simulink model "PV_Subsystem"  (R2024b)
settings: Solver=VariableStepAuto  StartTime=0.0  StopTime=10.0  RelTol=1e-3
libraries: spsSeriesRLCBranchLib x3, spsVoltageMeasurementLib x2, spsCurrentMeasurementLib x1, spsDiodeLib x1, spsIGBTDiodeLib x1, spsPVArrayLib x1, spsPWMGeneratorDCDCLib x1, sps_lib x1
settings Model: Creator=Raju  LastModifiedBy=Raju

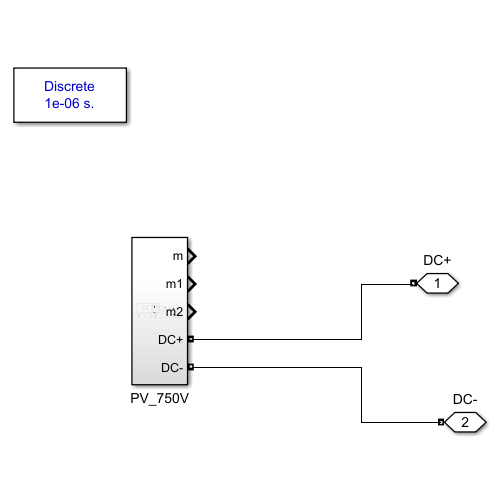
[thumbnail: Simulink's stored preview of the top-level diagram]
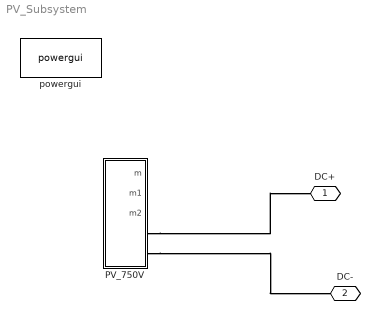
== system PV_Subsystem ==
  PV_750V : Subsystem
  powergui : sps_lib/powergui  Priority=1  SimulationMode=Discrete  SampleTime=1e-6  frequency=60  Iterations=50  frequencyindice=0  Pbase=100e6  ErrMax=1e-4  UnitsV=kV  UnitsW=MW  buscounter=0  FunctionMessages=off  echomessages=off  EnableUseOfTLC=off  CurrentSourceSwitches=off  DisableSnubberDevices=off  DisableRonSwitches=off  DisableVfSwitches=off  DisplayEquations=off  AutomaticDiscreteSolvers=off  SolverType=Tustin/Backward Euler (TBE)  Interpol=off  ExternalGateDelay=off  methode=off  Ts=100  x0status=blocks  SPID=on  SwTol=0  HookPort=off  NonlinearTolerance=1e-4  nMaxIteration=100  ContinueOnMaxIteration=off  RestoreLinks=warning  ResistiveCurrentMeasurement=off  Frange=[0:2:500]  Ylog=off  Xlog=on  ShowGrid=off  save=off  variable=ZData  structure=0  ZoomFFT=off  StartTime=0.0  cycles=1  DisplayStyle=1  fundamental=60  FreqAxis=off  MaxFrequency=1000  frequencyindicesteady=1  RmsSteady=1  display=off
  DC+ : PMIOPort  Side=Right
  DC- : PMIOPort  Port=2  Side=Right
  connections:
  PV_750V/RConn1 -- DC+/RConn1
  PV_750V/RConn2 -- DC-/RConn1

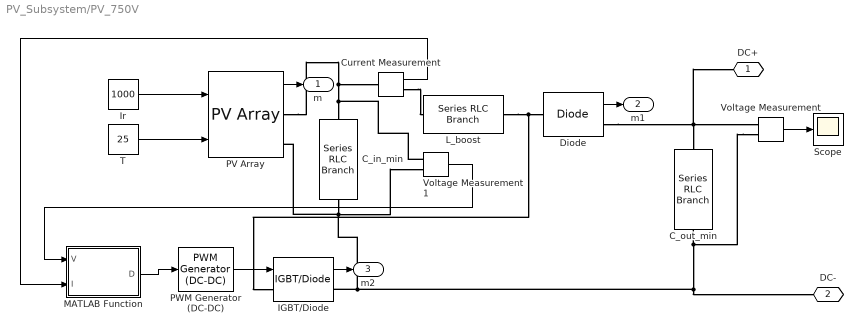
== system PV_Subsystem/PV_750V ==
  C_in_min : spsSeriesRLCBranchLib/Series RLC Branch  LConnTagsString=__new0  RConnTagsString=__new0  BranchType=C  Resistance=1  Inductance=1e-3  SetiL0=off  InitialCurrent=0  Capacitance=255e-6  Setx0=off  InitialVoltage=0  Measurements=None
  C_out_min : spsSeriesRLCBranchLib/Series RLC Branch  LConnTagsString=__new0  RConnTagsString=__new0  BranchType=C  Resistance=1  Inductance=1e-3  SetiL0=off  InitialCurrent=0  Capacitance=1208.2e-6  Setx0=off  InitialVoltage=0  Measurements=None
  Current Measurement : spsCurrentMeasurementLib/Current Measurement  PhasorSimulation=off  OutputType=Complex  PSBequivalent=0
  Diode : spsDiodeLib/Diode  Ron=0.001  Lon=0  Vf=0.8  IC=0  UseSnubber=0  Rs=500  Cs=250e-9  Measurements=on
  IGBT/Diode : spsIGBTDiodeLib/IGBT//Diode  Ron=1e-3  Rs=1e5  Cs=inf  Measurements=on
  Ir : Constant  Value=1000
  L_boost : spsSeriesRLCBranchLib/Series RLC Branch  LConnTagsString=__new0  RConnTagsString=__new0  BranchType=L  Resistance=1  Inductance=0.842e-3  SetiL0=off  InitialCurrent=0  Capacitance=1e-6  Setx0=off  InitialVoltage=0  Measurements=None
  MATLAB Function : MATLAB Function  TreatAsAtomicUnit=on
  PV Array : spsPVArrayLib/PV Array  Npar=36  Nser=9  PlotType=array @ 1000 W/m2 & specified temperatures  S_vec="[ 1000  500  100 ]"  Temp_C_vec="[ 45 25  ]"  ModuleName=User-defined  PlotWhenSelected=off  Pm=305.226  Ncell=96  Voc=64.20  Isc=5.96  Vm=54.70  Im=5.58  beta_Voc_pc=-0.36099  alpha_Isc_pc=0.102  beta_Voc=-0.23176  alpha_Isc=0.0060792  IL=5.9627  I0=2.2149e-10  nI=1.0848  Rsh=517.7141  Rs=0.23659  RobustModel=off  RobustCellTemperature=313.3991  BAL=on  Tc=1e-6  Tfilter=5e-5
  PWM Generator (DC-DC) : spsPWMGeneratorDCDCLib/PWM Generator (DC-DC)  Fsw=5000  Ts=0
  Scope : Scope
  T : Constant  Value=25
  Voltage Measurement : spsVoltageMeasurementLib/Voltage Measurement  PhasorSimulation=off  OutputType=Complex  PSBequivalent=0
  Voltage Measurement1 : spsVoltageMeasurementLib/Voltage Measurement  PhasorSimulation=off  OutputType=Complex  PSBequivalent=0
  DC+ : PMIOPort  Side=Right
  DC- : PMIOPort  Port=2  Side=Right
  m : Outport
  m1 : Outport  Port=2
  m2 : Outport  Port=3
  wires:
  MATLAB Function/1(D) -> PWM Generator (DC-DC)/1
  Current Measurement/1 -> MATLAB Function/2(I)
  PWM Generator (DC-DC)/1 -> IGBT/Diode/1
  Ir/1 -> PV Array/1
  Diode/1 -> m1/1
  Voltage Measurement1/1 -> MATLAB Function/1(V)
  T/1 -> PV Array/2
  Voltage Measurement/1 -> Scope/1
  IGBT/Diode/1 -> m2/1
  PV Array/1 -> m/1
  connections:
  Voltage Measurement/LConn2 -- DC-/RConn1 -- PV Array/RConn2 -- Voltage Measurement1/LConn2 -- C_in_min/RConn1 -- IGBT/Diode/RConn1 -- C_out_min/RConn1
  Current Measurement/RConn1 -- L_boost/LConn1
  Diode/RConn1 -- DC+/RConn1 -- Voltage Measurement/LConn1 -- C_out_min/LConn1
  PV Array/RConn1 -- Voltage Measurement1/LConn1 -- C_in_min/LConn1 -- Current Measurement/LConn1
  L_boost/RConn1 -- IGBT/Diode/LConn1 -- Diode/LConn1

== matlab function PV_Subsystem/PV_750V/MATLAB Function ==
  data: V input; D output; I input
function D = MPPT_PO(V, I)
persistent Vprev Pprev Dprev
if isempty(Vprev)
    Vprev = 0; Pprev = 0; Dprev = 0.55;
end
deltaD = 1e-4;
P = V * I;
dV = V - Vprev;
dP = P - Pprev;
if dP ~= 0
    if dP > 0
        if dV > 0
            D = Dprev - deltaD;
        else
            D = Dprev + deltaD;
        end
    else
        if dV > 0
            D = Dprev + deltaD;
        else
            D = Dprev - deltaD;
        end
    end
else
    D = Dprev;
end
D = min(max(D, 0.1), 0.85);
Vprev = V; Pprev = P; Dprev = D;
